simulink model "AE4311_CABS_CIBS"  (R2025a)
settings: Solver=FixedStepDiscrete  StartTime=0  StopTime=60  FixedStep=0.01  RelTol=1e-3
values from neighbouring files (symbols this model uses):
  cabsAdaptationOn = 0    [init_AE4311_simulink.m]
  cabsRho0 = rhoPerfect    [init_AE4311_simulink.m]
  controllerMode = 2    [init_AE4311_simulink.m]
  thetaCtrlSim = thetaTrue    [init_AE4311_simulink.m]
  thetaPlantSim = (1 + epsilon)*thetaTrue    [init_AE4311_simulink.m]
settings Model: Creator=erdem  LastModifiedBy=erdem

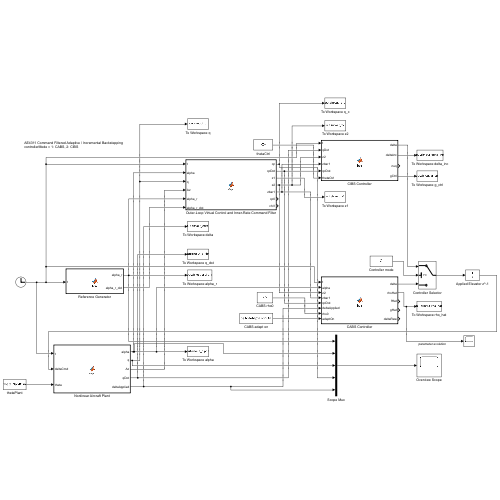
[thumbnail: Simulink's stored preview of the top-level diagram]
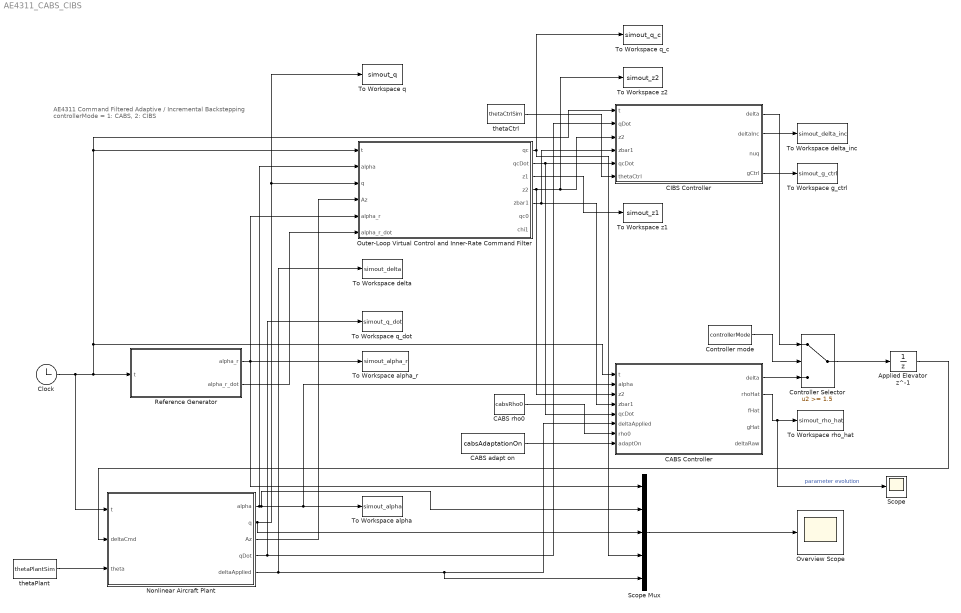
== system AE4311_CABS_CIBS ==
  note: AE4311 Command Filtered Adaptive / Incremental Backstepping
      | controllerMode = 1: CABS, 2: CIBS
  Applied Elevator z^-1 : UnitDelay  SampleTime=0.01  HasFrameUpgradeWarning=on
  CABS Controller : MATLAB Function  TreatAsAtomicUnit=on
  CABS adapt on : Constant  Value=cabsAdaptationOn
  CABS rho0 : Constant  Value=cabsRho0
  CIBS Controller : MATLAB Function  TreatAsAtomicUnit=on
  Clock : Clock
  Controller Selector : Switch  Threshold=1.5  SaturateOnIntegerOverflow=off  InputSameDT=off
  Controller mode : Constant  Value=controllerMode
  Nonlinear Aircraft Plant : MATLAB Function  TreatAsAtomicUnit=on
  Outer-Loop Virtual Control and Inner-Rate Command Filter : MATLAB Function  TreatAsAtomicUnit=on
  Overview Scope : Scope
      settings: ActiveDisplayYMinimum=-1  ActiveDisplayYMaximum=1
  Reference Generator : MATLAB Function  TreatAsAtomicUnit=on
  Scope : Scope
      settings: ActiveDisplayYMinimum=0.682408489751219  ActiveDisplayYMaximum=1.3583235922390289
  Scope Mux : Mux  Inputs=5
  To Workspace alpha : ToWorkspace  VariableName=simout_alpha  SaveFormat=Timeseries  SampleTime=-1
  To Workspace alpha_r : ToWorkspace  VariableName=simout_alpha_r  SaveFormat=Timeseries  SampleTime=-1
  To Workspace delta : ToWorkspace  VariableName=simout_delta  SaveFormat=Timeseries  SampleTime=-1
  To Workspace delta_inc : ToWorkspace  VariableName=simout_delta_inc  SaveFormat=Timeseries  SampleTime=-1
  To Workspace g_ctrl : ToWorkspace  VariableName=simout_g_ctrl  SaveFormat=Timeseries  SampleTime=-1
  To Workspace q : ToWorkspace  VariableName=simout_q  SaveFormat=Timeseries  SampleTime=-1
  To Workspace q_c : ToWorkspace  VariableName=simout_q_c  SaveFormat=Timeseries  SampleTime=-1
  To Workspace q_dot : ToWorkspace  VariableName=simout_q_dot  SaveFormat=Timeseries  SampleTime=-1
  To Workspace rho_hat : ToWorkspace  VariableName=simout_rho_hat  SaveFormat=Timeseries  SampleTime=-1
  To Workspace z1 : ToWorkspace  VariableName=simout_z1  SaveFormat=Timeseries  SampleTime=-1
  To Workspace z2 : ToWorkspace  VariableName=simout_z2  SaveFormat=Timeseries  SampleTime=-1
  thetaCtrl : Constant  Value=thetaCtrlSim
  thetaPlant : Constant  Value=thetaPlantSim
  wires:
  Reference Generator/2(alpha_r_dot) -> Outer-Loop Virtual Control and Inner-Rate Command Filter/6(alpha_r_dot)
  Clock/1 -> CIBS Controller/1(t), Outer-Loop Virtual Control and Inner-Rate Command Filter/1(t), CABS Controller/1(t), Reference Generator/1(t), Nonlinear Aircraft Plant/1(t)
  thetaPlant/1 -> Nonlinear Aircraft Plant/3(theta)
  Reference Generator/1(alpha_r) -> Outer-Loop Virtual Control and Inner-Rate Command Filter/5(alpha_r), To Workspace alpha_r/1, Scope Mux/1
  Nonlinear Aircraft Plant/1(alpha) -> To Workspace alpha/1, CABS Controller/2(alpha), Scope Mux/2, Outer-Loop Virtual Control and Inner-Rate Command Filter/2(alpha)
  Nonlinear Aircraft Plant/4(qDot) -> CIBS Controller/2(qDot), To Workspace q_dot/1
  Nonlinear Aircraft Plant/3(Az) -> Outer-Loop Virtual Control and Inner-Rate Command Filter/4(Az)
  Nonlinear Aircraft Plant/2(q) -> Outer-Loop Virtual Control and Inner-Rate Command Filter/3(q), To Workspace q/1, Scope Mux/3
  Nonlinear Aircraft Plant/5(deltaApplied) -> CABS Controller/6(deltaApplied), Scope Mux/5, To Workspace delta/1
  CABS adapt on/1 -> CABS Controller/8(adaptOn)
  thetaCtrl/1 -> CIBS Controller/6(thetaCtrl)
  Outer-Loop Virtual Control and Inner-Rate Command Filter/1(qc) -> To Workspace q_c/1, Scope Mux/4
  Outer-Loop Virtual Control and Inner-Rate Command Filter/2(qcDot) -> CABS Controller/5(qcDot), CIBS Controller/5(qcDot)
  Outer-Loop Virtual Control and Inner-Rate Command Filter/3(z1) -> To Workspace z1/1
  Outer-Loop Virtual Control and Inner-Rate Command Filter/4(z2) -> CIBS Controller/3(z2), To Workspace z2/1, CABS Controller/3(z2)
  CABS Controller/1(delta) -> Controller Selector/3
  Outer-Loop Virtual Control and Inner-Rate Command Filter/5(zbar1) -> CABS Controller/4(zbar1), CIBS Controller/4(zbar1)
  Controller mode/1 -> Controller Selector/2
  CABS rho0/1 -> CABS Controller/7(rho0)
  CIBS Controller/1(delta) -> Controller Selector/1
  CIBS Controller/2(deltaInc) -> To Workspace delta_inc/1
  CIBS Controller/4(gCtrl) -> To Workspace g_ctrl/1
  CABS Controller/2(rhoHat) -> Scope/1, To Workspace rho_hat/1  "parameter evolution"
  Applied Elevator z^-1/1 -> Nonlinear Aircraft Plant/2(deltaCmd)
  Scope Mux/1 -> Overview Scope/1
  Controller Selector/1 -> Applied Elevator z^-1/1

== matlab function AE4311_CABS_CIBS/Outer-Loop Virtual Control and Inner-Rate Command Filter ==
  data: t input; qc output; alpha input; q input; Az input; alpha_r input; alpha_r_dot input; qcDot output; z1 output; z2 output; zbar1 output; qc0 output; chi1 output
function [qc,qcDot,z1,z2,zbar1,qc0,chi1] = ...
    fcn(t,alpha,q,Az,alpha_r,alpha_r_dot)

persistent xcf chi

if isempty(xcf) || t <= 0
    xcf = [0;0];
    chi = 0;
end

% Controller parameters
c1 = 4;
VT = 3109.3;
Ts = 0.01;

% Tracking error
z1 = alpha - alpha_r;

% Raw virtual pitch-rate command
qc0 = -c1*z1 - Az/VT + alpha_r_dot;

% Discrete second-order command filter
A11 = 0.981803;
A12 = 0.00866405;
A21 = -3.46562;
A22 = 0.739209;

B1 = 0.0181974;
B2 = 3.46562;

x1 = A11*xcf(1) + A12*xcf(2) + B1*qc0;
x2 = A21*xcf(1) + A22*xcf(2) + B2*qc0;

xcf = [x1;x2];

qc    = xcf(1);
qcDot = xcf(2);

% Command-filter compensation
chi = chi + Ts*(-c1*chi + (qc - qc0));

chi1  = chi;
zbar1 = z1 - chi1;

% Inner-loop tracking error
z2 = q - qc;
end

== matlab function AE4311_CABS_CIBS/Reference Generator ==
  data: t input; alpha_r output; alpha_r_dot output
function [alpha_r,alpha_r_dot] = fcn(t)

% Reference:
% alpha_r = 11 deg * sin(0.6 t)

alphaAmp = 0.191986;
omegaRef = 0.6;

alpha_r = alphaAmp*sin(omegaRef*t);

alpha_r_dot = alphaAmp*omegaRef*cos(omegaRef*t);

end

== matlab function AE4311_CABS_CIBS/CABS Controller ==
  data: t input; delta output; alpha input; z2 input; zbar1 input; qcDot input; deltaApplied input; rho0 input; adaptOn input; rhoHat output; fHat output; gHat output; deltaRaw output
function [delta,rhoHat,fHat,gHat,deltaRaw] = ...
    fcn(t,alpha,z2,zbar1,qcDot,deltaApplied,rho0,adaptOn)

persistent rho

if isempty(rho) || t <= 0
    rho = rho0;
end

% Parameters
M    = 2.2;
Kq   = 11.08945;
Ts   = 0.01;
c2   = 8;

dmax = 0.165806;
gmin = 20;

% Nominal aerodynamic parameter vector
tNom = [ ...
     303.1;
    -246.3;
     -37.56;
      71.51;
      10.01;
      12.0393;
      48.2246];

% Adaptation gains
G = [ ...
    0.02;
    0.02;
    0.02;
    0.02;
    0.02;
    0.0005;
    0.0005];

% Parameter bounds
rmin = 0.4*ones(7,1);
rmax = 1.6*ones(7,1);

% Parameter reconstruction
tHat = tNom .* rho;

% Regressors
aa = alpha*abs(alpha);

Yf = Kq*[ ...
    alpha^3, ...
    aa, ...
    alpha, ...
    M*aa, ...
    M*alpha];

Yg = Kq*[M,1];

% Estimated nonlinear dynamics
fHat = Yf*tHat(1:5);
gHat = Yg*tHat(6:7);

% Avoid singular inversion
if abs(gHat) < gmin
    if gHat >= 0
        gHat = gmin;
    else
        gHat = -gmin;
    end
end

% CABS control law
deltaRaw = (qcDot - c2*z2 - zbar1 - fHat)/gHat;
% Saturation
delta = min(max(deltaRaw,-dmax),dmax);
isSat = abs(deltaRaw) > dmax;

%% Adaptive update

if adaptOn > 0.5 && ~isSat
    Yfull = [Yf, Yg*deltaApplied];
    Psi = Yfull .* tNom.';
    rhoDot = G .* (Psi.'*z2);
    % Projection logic
    for i = 1:7
        if rho(i) <= rmin(i) && rhoDot(i) < 0
            rhoDot(i) = 0;
        elseif rho(i) >= rmax(i) && rhoDot(i) > 0
            rhoDot(i) = 0;
        end
    end
    rho = rho + Ts*rhoDot;
    rho = min(max(rho,rmin),rmax);
end
rhoHat = rho;
end

== matlab function AE4311_CABS_CIBS/CIBS Controller ==
  data: t input; delta output; qDot input; z2 input; zbar1 input; qcDot input; thetaCtrl input; deltaInc output; nuq output; gCtrl output
function [delta,deltaInc,nuq,gCtrl] = ...
    fcn(t,qDot,z2,zbar1,qcDot,thetaCtrl)

persistent deltaPrev

if isempty(deltaPrev) || t <= 0
    deltaPrev = 0;
end

% Parameters
M    = 2.2;
Kq   = 11.08945;
c2   = 8;
dmax = 0.165806;

% Nominal control effectiveness
gCtrl = Kq*(thetaCtrl(6)*M + thetaCtrl(7));

% Desired angular acceleration
nuq = qcDot - c2*z2 - zbar1;

% Incremental elevator command
deltaInc = (nuq - qDot)/gCtrl;

% Total elevator command
deltaRaw = deltaPrev + deltaInc;

% Actuator saturation
delta = min(max(deltaRaw,-dmax),dmax);

% Store previous command
deltaPrev = delta;

end

== matlab function AE4311_CABS_CIBS/Nonlinear Aircraft Plant ==
  data: t input; alpha output; deltaCmd input; theta input; q output; Az output; qDot output; deltaApplied output
function [alpha,q,Az,qDot,deltaApplied] = ...
    fcn(t,deltaCmd,theta)

persistent x

if isempty(x) || t <= 0
    x = [0;0];
end

% Simulation and aircraft parameters
Ts   = 0.01;
M    = 2.2;
qbar = 6132.8;
S    = 0.44;
m    = 13.9752;
VT   = 3109.3;
Kq   = 11.08945;

% Current measured outputs
alpha = x(1);
q     = x(2);

% Applied elevator
deltaApplied = deltaCmd;

%% Current aerodynamic quantities

aa = alpha*abs(alpha);

phiZ1 = -288.7*alpha^3 + 50.32*aa - 23.89*alpha;

phiZ2 = -13.53*aa +4.185*alpha;

Cz = phiZ1 + M*phiZ2;

bz = 1.6238*M - 6.7240;

Az = (qbar*S/m)*(Cz + bz*deltaCmd);

Yf = Kq*[ ...
    alpha^3, ...
    aa, ...
    alpha, ...
    M*aa, ...
    M*alpha];

Yg = Kq*[M,1];

qDot = Yf*theta(1:5) + (Yg*theta(6:7))*deltaCmd;


%% RK4 stage 1

a1 = x(1);
q1 = x(2);

aa1 = a1*abs(a1);

phiZ11 = -288.7*a1^3 + 50.32*aa1 - 23.89*a1;

phiZ21 = -13.53*aa1 + 4.185*a1;

Cz1 = phiZ11 + M*phiZ21;

Az1 = (qbar*S/m)*(Cz1 + bz*deltaCmd);

k1a = q1 + Az1/VT;

Yf1 = Kq*[ ...
    a1^3, ...
    aa1, ...
    a1, ...
    M*aa1, ...
    M*a1];

k1q = Yf1*theta(1:5) + (Yg*theta(6:7))*deltaCmd;


%% RK4 stage 2

a2 = x(1) + 0.5*Ts*k1a;
q2 = x(2) + 0.5*Ts*k1q;

aa2 = a2*abs(a2);

phiZ12 = ...
    -288.7*a2^3 ...
    +50.32*aa2 ...
    -23.89*a2;

phiZ22 = ...
    -13.53*aa2 ...
    +4.185*a2;

Cz2 = phiZ12 + M*phiZ22;

Az2 = ...
    (qbar*S/m)*(Cz2 + bz*deltaCmd);

k2a = ...
    q2 + Az2/VT;

Yf2 = Kq*[ ...
    a2^3, ...
    aa2, ...
    a2, ...
    M*aa2, ...
    M*a2];

k2q = ...
    Yf2*theta(1:5) ...
    + (Yg*theta(6:7))*deltaCmd;


%% RK4 stage 3

a3 = x(1) + 0.5*Ts*k2a;
q3 = x(2) + 0.5*Ts*k2q;

aa3 = a3*abs(a3);

phiZ13 = ...
    -288.7*a3^3 ...
    +50.32*aa3 ...
    -23.89*a3;

phiZ23 = ...
    -13.53*aa3 ...
    +4.185*a3;

Cz3 = phiZ13 + M*phiZ23;

Az3 = ...
    (qbar*S/m)*(Cz3 + bz*deltaCmd);

k3a = ...
    q3 + Az3/VT;

Yf3 = Kq*[ ...
    a3^3, ...
    aa3, ...
    a3, ...
    M*aa3, ...
    M*a3];

k3q = ...
    Yf3*theta(1:5) ...
    + (Yg*theta(6:7))*deltaCmd;


%% RK4 stage 4

a4 = x(1) + Ts*k3a;
q4 = x(2) + Ts*k3q;

aa4 = a4*abs(a4);

phiZ14 = ...
    -288.7*a4^3 ...
    +50.32*aa4 ...
    -23.89*a4;

phiZ24 = ...
    -13.53*aa4 ...
    +4.185*a4;

Cz4 = phiZ14 + M*phiZ24;

Az4 = ...
    (qbar*S/m)*(Cz4 + bz*deltaCmd);

k4a = ...
    q4 + Az4/VT;

Yf4 = Kq*[ ...
    a4^3, ...
    aa4, ...
    a4, ...
    M*aa4, ...
    M*a4];

k4q = ...
    Yf4*theta(1:5) ...
    + (Yg*theta(6:7))*deltaCmd;


%% Advance x_k -> x_{k+1}

x = x + Ts/6 * [ ...
    k1a + 2*k2a + 2*k3a + k4a;
    k1q + 2*k2q + 2*k3q + k4q];

end
